simulink model "residual_FWD_INV_validation_v2"  (R2025a)
settings: Solver=VariableStepAuto  StartTime=0.0  StopTime=212  RelTol=1e-3
undefined symbols (not defined in the file or in its folder): National_Instruments, PCI, shadowInverseOptions, shadowOptions, shadowPressureOptions, singlePassOptions
libraries: sldrtlib x3
(part 1 of 2)
settings Model: Creator=dperera  LastModifiedBy=dperera

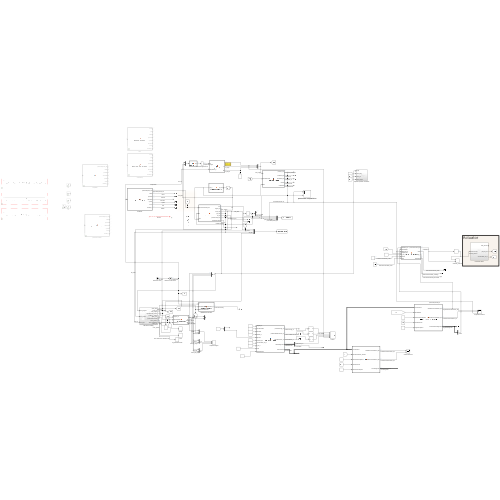
[thumbnail: Simulink's stored preview of the top-level diagram]
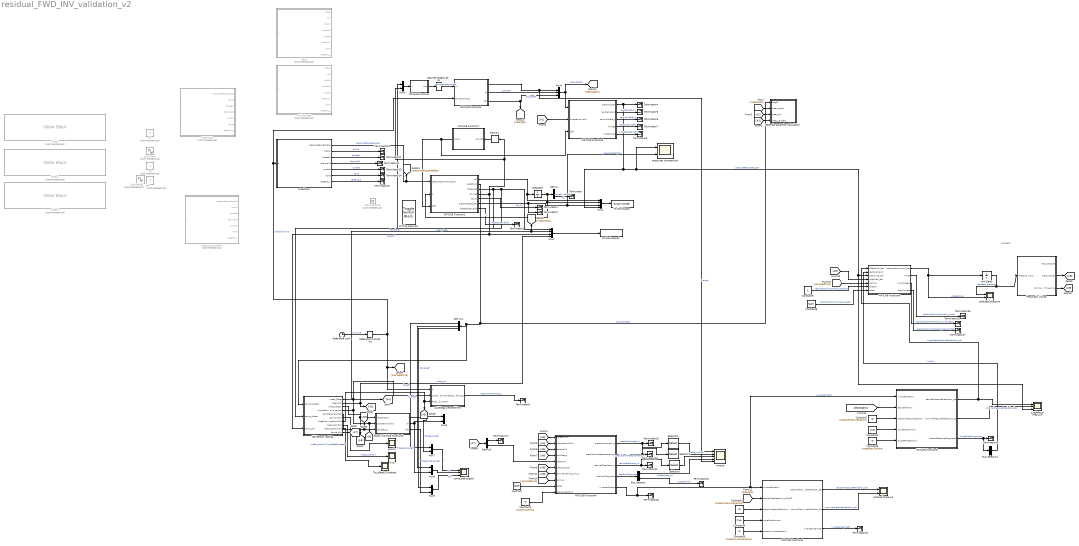
== system residual_FWD_INV_validation_v2 ==
  note: Actuator
  Bus Selector : BusSelector  OutputSignals=qMeasured_m,scoreValid
  Bus Selector1 : BusSelector  OutputSignals=valid
  Constant : Constant  Value=false  OutDataTypeStr=boolean
  Constant1 : Constant  Value=shadowOptions
  Constant2 : Constant  Value=shadowPressureOptions
  Constant3 : Constant  Value=shadowInverseOptions
  Constant4 : Constant  Value=true  OutDataTypeStr=boolean
  Constant5 : Constant  Value=true  OutDataTypeStr=boolean
  Constant6 : Constant  Value=singlePassOptions
  Constant7 : Constant  Value=shadowPressureOptions
  Constant8 : Constant  Value=false  OutDataTypeStr=boolean
  Constant9 : Constant
  Demux : Demux  Outputs=2
  Demux1 : Demux  Outputs=3
  Demux2 : Demux  Outputs=2
  Desired lengths 50 ms : ZeroOrderHold  SampleTime=0.05
  Integrator : Integrator  InitialCondition=[0;0;0;0]
  Inverse : Scope  NumInputPorts=5
      settings: ActiveDisplayYMinimum=-0.047306176084099816  ActiveDisplayYMaximum=0.024967148488830526  DataLoggingVariableName=ScopeData12
  MATLAB Function : MATLAB Function  TreatAsAtomicUnit=on
  MATLAB Function1 : MATLAB Function  TreatAsAtomicUnit=on
  MATLAB Function2 : MATLAB Function  TreatAsAtomicUnit=on
  MATLAB Function3 : MATLAB Function  TreatAsAtomicUnit=on
  MATLAB Function4 : MATLAB Function  TreatAsAtomicUnit=on
  MATLAB Function5 : MATLAB Function  TreatAsAtomicUnit=on
  MATLAB Function6 : MATLAB Function  TreatAsAtomicUnit=on
  MATLAB Function7 : MATLAB Function  TreatAsAtomicUnit=on
  MATLAB Function8 : MATLAB Function  TreatAsAtomicUnit=on
  MATLAB Function9 : MATLAB Function  TreatAsAtomicUnit=on
  Memory : Memory  InitialCondition=0.01
  Mux1 : Mux
  Mux2 : Mux
  Mux{3,5,7..9} (5 alike) : Mux  Inputs=2
  Mux6 : Mux  Inputs=3
  NDI Sensor reading : Subsystem
  P1 : Constant  Commented=on  Value=0
  P2 : Constant  Commented=on  Value=0
  P3 : Constant  Commented=on  Value=0
  Pneumatic Valves : Subsystem
  Reference clock : Clock
  Reference time 50 ms : ZeroOrderHold  SampleTime=0.05
  Selector1 : Selector  NumberOfDimensions=2  InputPortWidth=3  IndexOptions=Select all,Index vector (dialog)  Indices=[1 3],1  OutputSizes=1,1
  Selector2 : Selector  NumberOfDimensions=2  InputPortWidth=3  IndexOptions=Select all,Index vector (dialog)  Indices=[1 3],1  OutputSizes=1,1
  Selector3 : Selector  NumberOfDimensions=2  InputPortWidth=3  IndexOptions=Select all,Index vector (dialog)  Indices=[1 3],1  OutputSizes=1,1
  Seperate paramter calculation : Subsystem
  Sine Wave : Sin  Commented=on  Amplitude=1.5  Bias=1.5  Frequency=0.2  Phase=3*pi/2  SampleTime=0
  Sine Wave1 : Sin  Commented=on  Amplitude=1.5  Bias=1.5  Frequency=0.2  Phase=3*pi/2  SampleTime=0
  Slider : SliderBlock  Commented=on  ScaleMax=3
  Slider1 : SliderBlock  Commented=on  ScaleMax=3
  Slider2 : SliderBlock  Commented=on  ScaleMax=3
  Terminator{,1..15,17..27} (27 alike) : Terminator
  Terminator16 : Terminator  Commented=on
  Tip_offsetCOrrected : Scope
      settings: ActiveDisplayYMinimum=-0.22727653062343597  ActiveDisplayYMaximum=0.33693047368526458  DataLoggingVariableName=ScopeData9
  To Workspace : ToWorkspace  VariableName=dynamicModel  SaveFormat=Timeseries  SampleTime=-1
  To Workspace1 : ToWorkspace  VariableName=dynamic_NDI_meas_angle  SaveFormat=Timeseries  SampleTime=-1
  Unit Delay : UnitDelay  InitialCondition=[0;0;0]  SampleTime=0.05  HasFrameUpgradeWarning=on
  XYZ : Scope
      settings: ActiveDisplayYMinimum=-0.22727653062343597  ActiveDisplayYMaximum=0.33693047368526458  DataLoggingVariableName=ScopeData15
  circlesweep : MATLAB Function  Commented=on  TreatAsAtomicUnit=on
  computed lengths : Scope  NumInputPorts=3
      settings: ActiveDisplayYMinimum=-0.016802180124961048  ActiveDisplayYMaximum=0.019521084576218834  DataLoggingVariableName=ScopeData11
  gravity : Scope
      settings: ActiveDisplayYMinimum=-11.042014198482379  ActiveDisplayYMaximum=1.2784590278504426  DataLoggingVariableName=ScopeData10
  helix : MATLAB Function  Commented=on  TreatAsAtomicUnit=on
  kill the pressure : ToggleSwitchBlock
  pressure combine : MATLAB Function  Commented=on  TreatAsAtomicUnit=on
  pressures comparision : Scope  NumInputPorts=2
      settings: ActiveDisplayYMinimum=-0.37499999999999989  ActiveDisplayYMaximum=3.375  DataLoggingVariableName=ScopeData6
  residual Pressure : Scope  NumInputPorts=2
      settings: ActiveDisplayYMinimum=-0.44669940616060977  ActiveDisplayYMaximum=0.544979494551485  DataLoggingVariableName=ScopeData14
  selected_pressure : Scope  NumInputPorts=2
      settings: ActiveDisplayYMinimum=-0.37499999999999994  ActiveDisplayYMaximum=3.3750000000000004  DataLoggingVariableName=ScopeData17
  sineWave : MATLAB Function  TreatAsAtomicUnit=on
  singlePassl Pressure : Scope  NumInputPorts=3
      settings: ActiveDisplayYMinimum=-1.0880434782608694  ActiveDisplayYMaximum=2.9119565217391306  DataLoggingVariableName=ScopeData16
  stepWave : MATLAB Function  Commented=on  TreatAsAtomicUnit=on
  validMeasurementTime : MATLAB Function  TreatAsAtomicUnit=on
  wires:
  MATLAB Function1/1(dX) -> Mux1/1, Integrator/1  "dX"
  Integrator/1 -> MATLAB Function1/2(X), Mux1/2, Demux/1  "X"
  Demux/2 -> Terminator/1  "length velocity"
  MATLAB Function1/5(tau_N) -> Terminator1/1  "tau_N"
  MATLAB Function1/6(pressureUsed_bar) -> Terminator2/1, pressures comparision/2, Mux1/3  "pressureUsed_bar"
  MATLAB Function1/7(thetaObservable) -> Terminator3/1  "thetaObservable"
  Mux1/1 -> To Workspace/1
  Mux2/1 -> To Workspace1/1
  Mux6/1 -> MATLAB Function3/1(l), [deslengths]  "des_lengths"
  [A1] -> MATLAB Function3/2(orientationValid)
  MATLAB Function3/2(tauDesired_N) -> Terminator5/1  "tauDesired_N"
  MATLAB Function3/3(tauAvailable_N) -> Terminator6/1  "tauAvailable_N"
  MATLAB Function3/4(limited) -> Terminator7/1  "pressureLimited"
  MATLAB Function3/5(modelValid) -> Terminator8/1  "inverseModelValid"
  MATLAB Function7/1(k_N_m) -> MATLAB Function3/3(stiff), MATLAB Function1/3(stiff)
  Memory/1 -> MATLAB Function7/1(phi_rad)
  NDI Sensor reading/5(pollStart_s_control) -> MATLAB Function5/3(pollStart_s), [A6]
  NDI Sensor reading/8(meas_position) -> XYZ/1  "meas_position"
  NDI Sensor reading/1(meas_theta) -> [meastheta], Mux2/2  "meas_theta"
  NDI Sensor reading/3(meas_length) -> MATLAB Function5/1(lengths3_m), [A3]
  NDI Sensor reading/4(orientationValid_control) -> [A4], MATLAB Function5/2(orientationValid), validMeasurementTime/2(orientationValid), [A1]
  NDI Sensor reading/2(meas_phi) -> [A2], Mux2/4  "meas_phi"
  MATLAB Function5/1(l) -> Mux7/2, Mux5/1  "fitered_length"
  Demux1/3 -> Mux9/1  "dd_length"
  NDI Sensor reading/7(baseOreintationValid) -> [A5], validMeasurementTime/3(baseOrientationValid)
  Demux1/1 -> Mux7/1  "length"
  Demux1/2 -> Mux8/1  "d_length"
  Mux8/1 -> computed lengths/2  "dl"
  MATLAB Function5/3(ddl) -> Mux9/2  "filtered_dd_length"
  Mux7/1 -> computed lengths/1  "l"
  MATLAB Function5/2(dl) -> Mux8/2, Mux5/2  "filtered_d_length"
  Mux9/1 -> computed lengths/3  "ddl"
  [A3] -> Seperate paramter calculation/4(meas_lengths)
  [A2] -> Seperate paramter calculation/3(meas_phi)
  Reference clock/1 -> Reference time 50 ms/1  "sim time"
  Reference time 50 ms/1 -> MATLAB Function2/2(sampleTime_s), sineWave/1(t), [sampledtime], validMeasurementTime/1(t)  "sampled time"
  MATLAB Function1/2(lengths_m) -> Seperate paramter calculation/1(length), NDI Sensor reading/1(comp_lengths), Demux1/1  "comp_lengths"
  validMeasurementTime/1(measurementTime_s) -> Terminator9/1  "measurementTime_s"
  sineWave/2(trialId) -> Terminator10/1  "trialId"
  sineWave/3(phaseId) -> Terminator11/1  "phaseId"
  sineWave/4(channelId) -> Terminator12/1  "channelId"
  sineWave/5(cycleId) -> Terminator13/1  "cycleId"
  sineWave/6(done) -> Terminator14/1  "done"
  sineWave/7(testEnd_s) -> Terminator15/1  "testEnd_s"
  ? -> Terminator16/1  "direction"
  MATLAB Function/1(lout) -> Desired lengths 50 ms/1
  Desired lengths 50 ms/1 -> MATLAB Function2/1(lIn)  "sampled des_length"
  Mux3/1 -> MATLAB Function/1(u)
  MATLAB Function2/1(l) -> Inverse/5, Mux6/1  "length"
  MATLAB Function2/2(dl) -> Mux6/2  "d_length"
  MATLAB Function2/3(ddl) -> Mux6/3, [ddlength]  "dd_length"
  [meastheta] -> Seperate paramter calculation/2(meas_theta)
  NDI Sensor reading/9(meas_positionTip) -> Tip_offsetCOrrected/1  "meas_positionTip_offsetCorrected"
  NDI Sensor reading/6(gravity_arm) -> gravity/1
  MATLAB Function3/1(pressure_bar) -> Mux1/4, pressures comparision/1, MATLAB Function9/3(pNominal_bar), singlePassl Pressure/3, Terminator4/1  "pressureRequested_bar"
  [A3] -> MATLAB Function4/1(lengths3_m)
  [A4] -> MATLAB Function4/2(orientationValid)
  [A5] -> MATLAB Function4/3(baseValid)
  [A6] -> MATLAB Function4/4(pollStart_s)
  Demux2/2 -> MATLAB Function4/5(tipFrame)
  NDI Sensor reading/10(frame_out) -> [A7]
  [A7] -> Demux2/1
  Demux2/1 -> Terminator17/1
  [A8] -> MATLAB Function4/6(pressure_bar)
  [sampledtime] -> MATLAB Function4/8(t_sim_s)
  Constant/1 -> MATLAB Function4/9(reset)
  Constant1/1 -> MATLAB Function4/10(shadowOptions)
  Pneumatic Valves/2(pressure_bar) -> [A8]
  Pneumatic Valves/3(commandTime_sim_s) -> [A9]
  [A9] -> MATLAB Function4/7(commandTime_sim_s)
  MATLAB Function4/4(shadowDiagnostic) -> Bus Selector/1  "shadowDiagnotic"
  MATLAB Function4/5(inverseContext) -> MATLAB Function8/1(inverseContext), MATLAB Function6/1(inverseContext), Terminator18/1  "inverseContext"
  MATLAB Function4/1(predictionLength_m) -> Selector2/1, Terminator19/1  "predictionLength_m"
  MATLAB Function4/2(predictionAtMeasurement_m) -> Selector1/1, Terminator20/1  "predictionAtMeasurement_m"
  MATLAB Function4/3(retimedPrediction_m) -> Selector3/1, Terminator21/1  "retimePrediction_m"
  Bus Selector/1 -> Inverse/4  "<qMeasured_m>"
  Selector1/1 -> Inverse/2  "pred_withNDI"
  Bus Selector/2 -> Terminator22/1  "<scoreValid>"
  MATLAB Function1/3(theta_rad) -> NDI Sensor reading/2(comp_ltheta), Mux3/1, Mux2/1  "des_theta"
  MATLAB Function1/4(phi_rad) -> NDI Sensor reading/3(comp_phi), Mux2/3, Mux3/2, Memory/1  "des_phi"
  Selector2/1 -> Inverse/1
  Selector3/1 -> Inverse/3
  [ddlength] -> MATLAB Function6/2(desiredAcceleration_mPerS2)
  Constant2/1 -> MATLAB Function6/3(shadowPressureOptions)
  Constant3/1 -> MATLAB Function6/5(shadowInverseOptions)
  Constant4/1 -> MATLAB Function6/4(variableCommon)
  MATLAB Function6/3(inverseDiagnostic) -> Terminator23/1  "inverseDiagnostic"
  MATLAB Function6/1(residualPressurePrediction_bar) -> residual Pressure/1  "residualPressurePrediction_bar"
  MATLAB Function6/2(nominalPressurePrediction_bar) -> residual Pressure/2  "nominalPressurePrediction_bar"
  Constant5/1 -> MATLAB Function8/4(variableCommon)
  Constant6/1 -> MATLAB Function8/5(singlePassOptions)
  Constant7/1 -> MATLAB Function8/3(shadowPressureOptions)
  MATLAB Function8/3(desiredPressureDiagnostic) -> Bus Selector1/1, Terminator24/1  "singlePassDiagnostic"
  MATLAB Function8/1(desiredPressurePrediction_bar) -> MATLAB Function9/1(pResidual_bar), singlePassl Pressure/1  "singlePassPressurePrediction_bar"
  MATLAB Function8/2(nominalPressurePrediction_bar) -> singlePassl Pressure/2  "nominalPressurePrediction_bar"
  [deslengths] -> MATLAB Function8/2(desiredMotion)
  MATLAB Function9/1(pressureCommand_bar) -> Unit Delay/1, selected_pressure/2  "useResidual"
  Unit Delay/1 -> selected_pressure/1, Pneumatic Valves/1(Pressure input)  "selected_pressure"
  Bus Selector1/1 -> MATLAB Function9/2(residualValid)  "<valid>"
  sineWave/1(pressureRequest_bar) -> MATLAB Function1/1(pressureCommand_bar), [pressureRequestedbar]  "pressureRequested_bar"
  [A8] -> MATLAB Function9/4(pApplied_bar)
  [sampledtime] -> MATLAB Function9/5(t_sim_s)
  Constant8/1 -> MATLAB Function9/7(reset)  "residualCommandValid_reset"
  Constant9/1 -> MATLAB Function9/6(enable)  "residualCommandValid_enable"
  MATLAB Function9/2(mode) -> Terminator25/1  "residualCommandValid_mode"
  MATLAB Function9/3(invalidAge_s) -> Terminator26/1  "residualCommandValid_invalidAge"
  MATLAB Function9/4(slewLimited) -> Terminator27/1  "residualCommandValid_slewLimited"

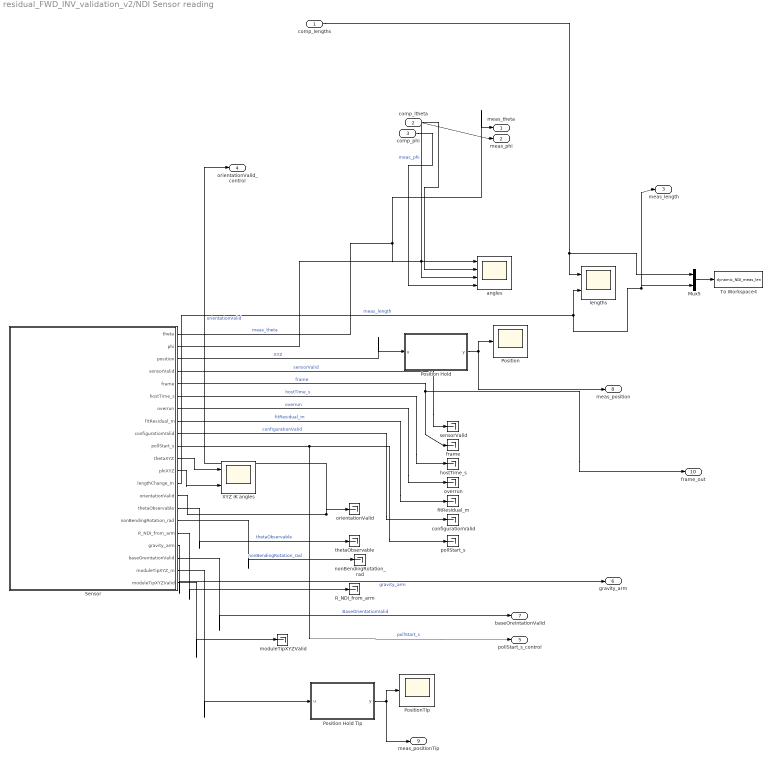
== system residual_FWD_INV_validation_v2/NDI Sensor reading ==
  comp_lengths : Inport
  comp_ltheta : Inport  Port=2
  comp_phi : Inport  Port=3
  Mux5 : Mux  Inputs=2
  Position : Scope
      settings: ActiveDisplayYMinimum=-0.21656345474719998  ActiveDisplayYMaximum=0.33777835857868188
  Position Hold : MATLAB Function  TreatAsAtomicUnit=on
  Position Hold Tip : MATLAB Function  TreatAsAtomicUnit=on
  PositionTip : Scope
      settings: ActiveDisplayYMinimum=-0.21656345474719998  ActiveDisplayYMaximum=0.33777835857868188  DataLoggingVariableName=ScopeData8
  R_NDI_from_arm : Terminator
  Sensor : Subsystem
  To Workspace4 : ToWorkspace  VariableName=dynamic_NDI_meas_len  SaveFormat=Timeseries  SampleTime=-1
  XYZ IK angles : Scope  NumInputPorts=2
      settings: DataLoggingVariableName=ScopeData2
  angles : Scope  NumInputPorts=4
      settings: ActiveDisplayYMinimum=-3.9269908169872414  ActiveDisplayYMaximum=3.9269908169872414
  configurationValid : Terminator
  fitResidual_m : Terminator
  frame : Terminator
  hostTime_s : Terminator
  lengths : Scope  NumInputPorts=2
      settings: ActiveDisplayYMinimum=-0.0017146774565175815  ActiveDisplayYMaximum=0.0020057370608089205  DataLoggingVariableName=ScopeData3
  moduleTipXYZValid : Terminator
  nonBendingRotation_rad : Terminator
  orientationValid : Terminator
  overrun : Terminator
  pollStart_s : Terminator
  sensorValid : Terminator
  thetaObservable : Terminator
  meas_theta : Outport
  meas_phi : Outport  Port=2
  meas_length : Outport  Port=3
  orientationValid_control : Outport  Port=4
  pollStart_s_control : Outport  Port=5
  gravity_arm : Outport  Port=6
  baseOreintationValid : Outport  Port=7
  meas_position : Outport  Port=8
  meas_positionTip : Outport  Port=9
  frame_out : Outport  Port=10
  wires:
  Sensor/13(lengthChange_m) -> lengths/2, meas_length/1, Mux5/2  "meas_length"
  comp_lengths/1 -> lengths/1, Mux5/1
  Sensor/10(pollStart_s) -> pollStart_s_control/1, pollStart_s/1  "pollStart_s"
  Sensor/2(phi) -> angles/3, meas_phi/1  "meas_phi"
  Sensor/3(position) -> Position Hold/1(u)  "XYZ"
  Sensor/1(theta) -> meas_theta/1, angles/1  "meas_theta"
  Sensor/6(hostTime_s) -> hostTime_s/1  "hostTIme_s"
  Sensor/9(configurationValid) -> configurationValid/1  "configurationValid"
  Sensor/4(sensorValid) -> sensorValid/1  "sensorValid"
  Sensor/7(overrun) -> overrun/1  "overrun"
  Sensor/5(frame) -> frame_out/1, frame/1  "frame"
  comp_ltheta/1 -> angles/2
  Sensor/8(fitResidual_m) -> fitResidual_m/1  "fitResidual_m"
  Sensor/12(phiXYZ) -> XYZ IK angles/2
  Sensor/11(thetaXYZ) -> XYZ IK angles/1
  Position Hold/1(y) -> Position/1, meas_position/1
  Mux5/1 -> To Workspace4/1
  Sensor/14(orientationValid) -> orientationValid_control/1, orientationValid/1  "orientationValid"
  Sensor/16(nonBendingRotation_rad) -> nonBendingRotation_rad/1  "nonBendingRotation_rad"
  Sensor/15(thetaObservable) -> thetaObservable/1  "thetaObservable"
  comp_phi/1 -> angles/4
  Sensor/19(baseOreintationValid) -> baseOreintationValid/1  "BaseOrientationValid"
  Sensor/17(R_NDI_from_arm) -> R_NDI_from_arm/1
  Sensor/18(gravity_arm) -> gravity_arm/1  "gravity_arm"
  Sensor/20(moduleTipXYZ_m) -> Position Hold Tip/1(u)
  Position Hold Tip/1(y) -> meas_positionTip/1, PositionTip/1
  Sensor/21(moduleTipXYZValid) -> moduleTipXYZValid/1

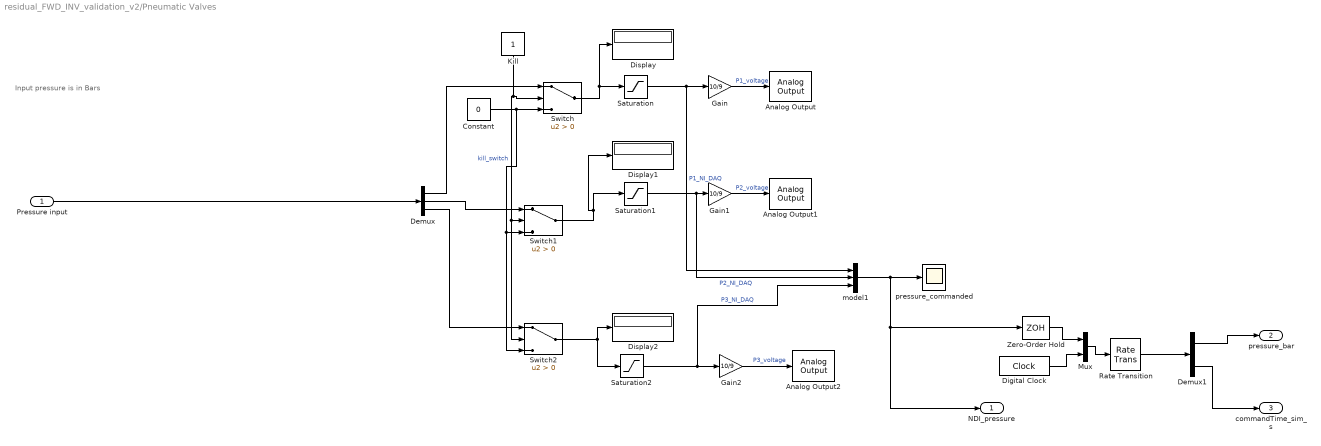
== system residual_FWD_INV_validation_v2/Pneumatic Valves ==
  note: Input pressure is in Bars
  Pressure input : Inport
  Analog Output : sldrtlib/Analog Output  SampleTime=1/100  MaxMissedTicks=inf  ShowMissedTicks=off  YieldWhenWaiting=off  DrvName=National_Instruments/PCI-6703  DrvAddress=4294967295  DrvOptions=0  Channels=1  RangeMode=1  VoltRange=1  InitialValue=0  FinalValue=0
      settings: AttributesFormatString=National Instruments\nPCI-6703 [auto]
  Analog Output1 : sldrtlib/Analog Output  SampleTime=1/100  MaxMissedTicks=inf  ShowMissedTicks=off  YieldWhenWaiting=off  DrvName=National_Instruments/PCI-6703  DrvAddress=4294967295  DrvOptions=0  Channels=2  RangeMode=1  VoltRange=1  InitialValue=0  FinalValue=0
      settings: AttributesFormatString=National Instruments\nPCI-6703 [auto]
  Analog Output2 : sldrtlib/Analog Output  SampleTime=1/100  MaxMissedTicks=inf  ShowMissedTicks=off  YieldWhenWaiting=off  DrvName=National_Instruments/PCI-6703  DrvAddress=4294967295  DrvOptions=0  Channels=3  RangeMode=1  VoltRange=1  InitialValue=0  FinalValue=0
      settings: AttributesFormatString=National Instruments\nPCI-6703 [auto]
  Constant : Constant  Value=0
  Demux : Demux  Outputs=3
  Demux1 : Demux  Outputs=[3 1]
  Digital Clock : DigitalClock  SampleTime=0.01
  Display : Display
  Display1 : Display
  Display2 : Display
  Gain : Gain  Gain=10/9
  Gain1 : Gain  Gain=10/9
  Gain2 : Gain  Gain=10/9
  Kill : Constant
  Mux : Mux  Inputs=2
  Rate Transition : RateTransition  InitialCondition=[0]  OutPortSampleTime=0.05
  Saturation : Saturate  UpperLimit=3  LowerLimit=0
  Saturation1 : Saturate  UpperLimit=3  LowerLimit=0
  Saturation2 : Saturate  UpperLimit=3  LowerLimit=0
  Switch : Switch  Criteria=u2 > Threshold  SaturateOnIntegerOverflow=off  InputSameDT=off
  Switch1 : Switch  Criteria=u2 > Threshold  SaturateOnIntegerOverflow=off  InputSameDT=off
  Switch2 : Switch  Criteria=u2 > Threshold  SaturateOnIntegerOverflow=off  InputSameDT=off
  Zero-Order Hold : ZeroOrderHold  SampleTime=0.01
  model1 : Mux  Inputs=3
  pressure_commanded : Scope
      settings: ActiveDisplayYMinimum=-0.37499999999999989  ActiveDisplayYMaximum=3.375  DataLoggingVariableName=ScopeData7
  NDI_pressure : Outport
  pressure_bar : Outport  Port=2
  commandTime_sim_s : Outport  Port=3
  wires:
  Constant/1 -> Switch2/3, Switch1/3, Switch/3
  Kill/1 -> Switch2/2, Switch1/2, Switch/2  "kill_switch"
  Switch/1 -> Display/1, Saturation/1
  Gain/1 -> Analog Output/1  "P1_voltage"
  Saturation/1 -> model1/1, Gain/1  "P1_NI_DAQ"
  Demux/3 -> Switch2/1
  Gain1/1 -> Analog Output1/1  "P2_voltage"
  Gain2/1 -> Analog Output2/1  "P3_voltage"
  Saturation2/1 -> model1/3, Gain2/1  "P3_NI_DAQ"
  Switch2/1 -> Saturation2/1, Display2/1
  Demux/2 -> Switch1/1
  Switch1/1 -> Saturation1/1, Display1/1
  model1/1 -> NDI_pressure/1, Zero-Order Hold/1, pressure_commanded/1
  Saturation1/1 -> model1/2, Gain1/1  "P2_NI_DAQ"
  Demux/1 -> Switch/1
  Pressure input/1 -> Demux/1
  Zero-Order Hold/1 -> Mux/1
  Digital Clock/1 -> Mux/2
  Mux/1 -> Rate Transition/1
  Rate Transition/1 -> Demux1/1
  Demux1/1 -> pressure_bar/1
  Demux1/2 -> commandTime_sim_s/1

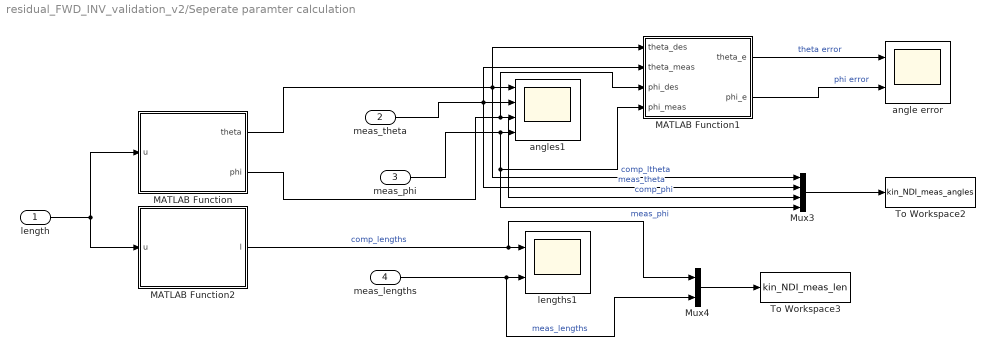
== system residual_FWD_INV_validation_v2/Seperate paramter calculation ==
  length : Inport
  meas_theta : Inport  Port=2
  meas_phi : Inport  Port=3
  meas_lengths : Inport  Port=4
  MATLAB Function : MATLAB Function  TreatAsAtomicUnit=on
  MATLAB Function1 : MATLAB Function  TreatAsAtomicUnit=on
  MATLAB Function2 : MATLAB Function  TreatAsAtomicUnit=on
  Mux3 : Mux
  Mux4 : Mux  Inputs=2
  To Workspace2 : ToWorkspace  VariableName=kin_NDI_meas_angles  SaveFormat=Timeseries  SampleTime=-1
  To Workspace3 : ToWorkspace  VariableName=kin_NDI_meas_len  SaveFormat=Timeseries  SampleTime=-1
  angle error : Scope  NumInputPorts=2
      settings: ActiveDisplayYMinimum=-3.908241267522468  ActiveDisplayYMaximum=3.9243412430226807  DataLoggingVariableName=ScopeData13
  angles1 : Scope  NumInputPorts=4
      settings: ActiveDisplayYMinimum=-3.9269137322662839  ActiveDisplayYMaximum=3.9265599408279468  DataLoggingVariableName=ScopeData4
  lengths1 : Scope  NumInputPorts=2
      settings: ActiveDisplayYMinimum=-0.02243223759551808  ActiveDisplayYMaximum=0.037530111947788623  DataLoggingVariableName=ScopeData5
  wires:
  meas_lengths/1 -> Mux4/2, lengths1/2  "meas_lengths"
  meas_theta/1 -> MATLAB Function1/2(theta_meas), Mux3/2, angles1/2  "meas_theta"
  MATLAB Function/2(phi) -> MATLAB Function1/3(phi_des), Mux3/3, angles1/3  "comp_phi"
  Mux3/1 -> To Workspace2/1
  meas_phi/1 -> MATLAB Function1/4(phi_meas), Mux3/4, angles1/4  "meas_phi"
  MATLAB Function/1(theta) -> MATLAB Function1/1(theta_des), Mux3/1, angles1/1  "comp_ltheta"
  Mux4/1 -> To Workspace3/1
  MATLAB Function2/1(l) -> Mux4/1, lengths1/1  "comp_lengths"
  length/1 -> MATLAB Function2/1(u), MATLAB Function/1(u)
  MATLAB Function1/1(theta_e) -> angle error/1  "theta error"
  MATLAB Function1/2(phi_e) -> angle error/2  "phi error"

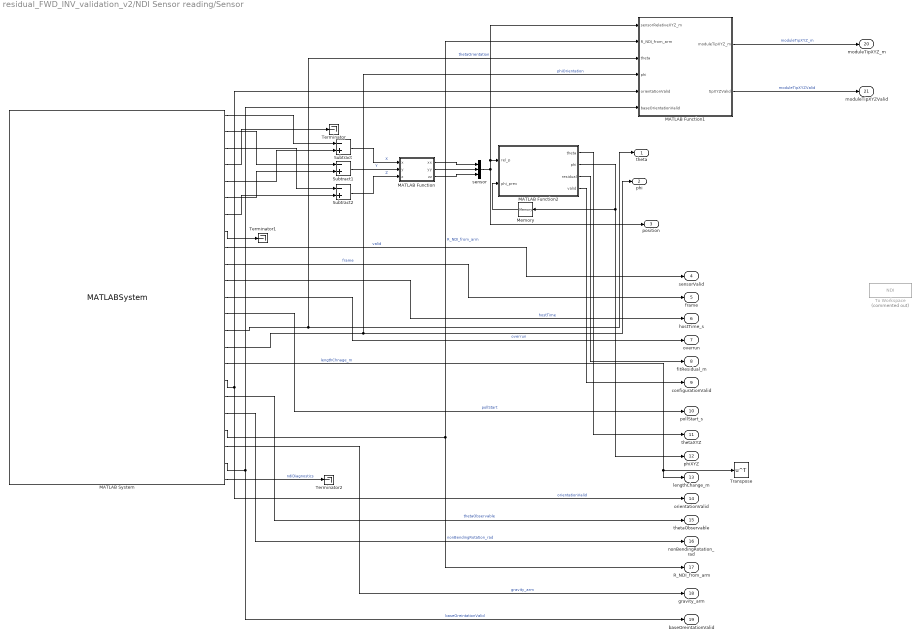
== system residual_FWD_INV_validation_v2/NDI Sensor reading/Sensor ==
  MATLAB Function : MATLAB Function  TreatAsAtomicUnit=on
  MATLAB Function1 : MATLAB Function  TreatAsAtomicUnit=on
  MATLAB Function2 : MATLAB Function  TreatAsAtomicUnit=on
  MATLAB System : MATLABSystem  System=AuroraReader_s2_BaseRotation  Port=COM12  BaudRate=921600  SamplePeriod=0.05  BaseSensorId=0A  TipSensorId=0B  CalibrationFile=C:\Users\dperera\OneDrive - Texas A&M University\Lab\Research\fDyn_ExpCom\hyDyn_Ctrl\ndi_orientation_recordings\calibration_20260930_190505_898.mat  PreflightSeconds=5  ActuatorRadius=0.013  ReferenceGravity_arm=[ 0; 0; -9.81 ]  SimulateUsing=Interpreted execution
      mask Type: AuroraReader_s2_BaseRotation
  Memory : Memory  InitialCondition=0.0001
  Subtract : Sum  Inputs=-+
  Subtract1 : Sum  Inputs=-+
  Subtract2 : Sum  Inputs=-+
  Terminator : Terminator
  Terminator1 : Terminator
  Terminator2 : Terminator
  To Workspace : ToWorkspace  Commented=on  VariableName=NDI  SaveFormat=Timeseries  SampleTime=-1
  Transpose : Math  Operator=transpose
  sensor : Mux  Inputs=3
  theta : Outport
  phi : Outport  Port=2
  position : Outport  Port=3
  sensorValid : Outport  Port=4
  frame : Outport  Port=5
  hostTime_s : Outport  Port=6
  overrun : Outport  Port=7
  fitResidual_m : Outport  Port=8
  configurationValid : Outport  Port=9
  pollStart_s : Outport  Port=10
  thetaXYZ : Outport  Port=11
  phiXYZ : Outport  Port=12
  lengthChange_m : Outport  Port=13
  orientationValid : Outport  Port=14
  thetaObservable : Outport  Port=15
  nonBendingRotation_rad : Outport  Port=16
  R_NDI_from_arm : Outport  Port=17
  gravity_arm : Outport  Port=18
  baseOreintationValid : Outport  Port=19
  moduleTipXYZ_m : Outport  Port=20
  moduleTipXYZValid : Outport  Port=21
  wires:
  MATLAB System/2 -> Subtract1/1
  MATLAB Function/3(zz) -> sensor/3
  Subtract1/1 -> MATLAB Function/2(y)  "Y"
  Subtract2/1 -> MATLAB Function/3(z)  "Z"
  MATLAB System/5 -> Subtract/2
  sensor/1 -> MATLAB Function1/1(sensorRelativeXYZ_m), MATLAB Function2/1(rel_p), position/1
  MATLAB System/8 -> Terminator1/1
  MATLAB Function/1(xx) -> sensor/1
  Subtract/1 -> MATLAB Function/1(x)  "X"
  MATLAB Function/2(yy) -> sensor/2
  MATLAB System/1 -> Subtract/1
  MATLAB Function2/2(phi) -> Memory/1, phiXYZ/1
  MATLAB System/7 -> Subtract2/2
  MATLAB System/4 -> Terminator/1
  MATLAB System/3 -> Subtract2/1
  MATLAB System/6 -> Subtract1/2
  Memory/1 -> MATLAB Function2/2(phi_prev)
  MATLAB System/9 -> sensorValid/1  "valid"
  MATLAB System/11 -> hostTime_s/1  "hostTime"
  MATLAB System/12 -> overrun/1  "overrun"
  MATLAB Function2/3(residual) -> fitResidual_m/1
  MATLAB Function2/4(valid) -> configurationValid/1
  MATLAB System/13 -> pollStart_s/1  "pollStart"
  MATLAB System/14 -> MATLAB Function1/3(theta), theta/1  "thetaOrientation"
  MATLAB System/15 -> MATLAB Function1/4(phi), phi/1  "phiOrientation"
  MATLAB Function2/1(theta) -> thetaXYZ/1
  MATLAB System/16 -> lengthChange_m/1, Transpose/1  "lengthChnage_m"
  MATLAB System/17 -> orientationValid/1, MATLAB Function1/5(orientationValid)  "orientationValid"
  MATLAB System/18 -> thetaObservable/1  "thetaObservable"
  MATLAB System/19 -> nonBendingRotation_rad/1  "nonBendingRotation_rad"
  MATLAB System/10 -> frame/1  "frame"
  MATLAB System/20 -> R_NDI_from_arm/1, MATLAB Function1/2(R_NDI_from_arm)  "R_NDI_from_arm"
  MATLAB System/21 -> gravity_arm/1  "gravity_arm"
  MATLAB System/22 -> baseOreintationValid/1, MATLAB Function1/6(baseOrientationValid)  "baseOreintationValid"
  MATLAB Function1/1(moduleTipXYZ_m) -> moduleTipXYZ_m/1  "moduleTipXYZ_m"
  MATLAB Function1/2(tipXYZValid) -> moduleTipXYZValid/1  "moduleTipXYZValid"
  MATLAB System/23 -> Terminator2/1  "ndiDiagnostics"

== matlab function residual_FWD_INV_validation_v2/validMeasurementTime ==
  data: t input; measurementTime_s output; orientationValid input; baseOrientationValid input
function measurementTime_s = validMeasurementTime( ...
    t, orientationValid, baseOrientationValid)
%#codegen

persistent lastValidTime
if isempty(lastValidTime)
    lastValidTime = -1.0;
end

if orientationValid && baseOrientationValid && isfinite(t)
    lastValidTime = t;
end

measurementTime_s = lastValidTime;
end

== matlab function residual_FWD_INV_validation_v2/NDI Sensor reading/Position Hold Tip ==
  data: u input; y output
function y = fcn(u)
persistent lastPosition
if isempty(lastPosition), lastPosition=nan(3,1); end
if all(isfinite(u)), lastPosition=u; end
y=lastPosition;
end

== matlab function residual_FWD_INV_validation_v2/MATLAB Function5 ==
  data: lengths3_m input; l output; dl output; ddl output; orientationValid input; pollStart_s input
function [l, dl, ddl] = filteredDerivatives(lengths3_m, orientationValid, pollStart_s)
%#codegen
% NDI lengths are [l1;l2;l3]; model coordinates are [l2;l3].
% Invalid or repeated BX frames do not update the derivative states.
persistent lastL lastT velocity acceleration
if isempty(lastT)
    lastL = nan(2,1);
    lastT = -1;
    velocity = zeros(2,1);
    acceleration = zeros(2,1);
end
l = lastL;
dl = velocity;
ddl = acceleration;
if ~orientationValid || ~all(isfinite(lengths3_m)) || ~isfinite(pollStart_s)
    return;
end
q = [lengths3_m(2); lengths3_m(3)];
if lastT < 0
    lastL = q;
    lastT = pollStart_s;
    l = q;
    return;
end
dt = pollStart_s-lastT;
if dt > 1e-6
    rawVelocity = (q-lastL)/dt;
    oldVelocity = velocity;
    alphaV = dt/(0.20+dt);
    velocity = velocity + alphaV*(rawVelocity-velocity);
    rawAcceleration = (velocity-oldVelocity)/dt;
    alphaA = dt/(0.30+dt);
    acceleration = acceleration + alphaA*(rawAcceleration-acceleration);
    lastL = q;
    lastT = pollStart_s;
end
l = lastL;
dl = velocity;
ddl = acceleration;
end

== matlab function residual_FWD_INV_validation_v2/sineWave ==
  data: t input; pressureRequest_bar output; trialId output; phaseId output; channelId output; cycleId output; done output; testEnd_s output
function [pressureRequest_bar,trialId,phaseId,channelId,cycleId,done,testEnd_s] = rlPressureSineBlock(t)
%#codegen
% OPEN-LOOP raw pressure request: peak/2*(1-cos(omega*time)).
% channelSelection: 1=P1, 2=P2, 3=P3, 0=all three separately.
channelSelection=0;
peak_bar=3.0;
omega_radPerS=0.8;
cyclesPerTrial=3;
repeats=2;
initialZero_s=5.0;
relax_s=10.0;
% phase: -1 invalid time, 0 initial zero, 4 zero relaxation,
% 5 periodic excitation, 9 complete. Cycles join at zero with zero slope.
assert(channelSelection>=0 && channelSelection<=3 && channelSelection==floor(channelSelection));
assert(peak_bar>=0 && peak_bar<=3 && omega_radPerS>0);
assert(cyclesPerTrial>=1 && cyclesPerTrial==floor(cyclesPerTrial));
assert(repeats>=1 && repeats==floor(repeats) && initialZero_s>=0 && relax_s>0);
nChannels=1;if channelSelection==0,nChannels=3;end
period_s=2*pi/omega_radPerS;
excitation_s=cyclesPerTrial*period_s;
trialDuration_s=excitation_s+relax_s;
nTrials=nChannels*repeats;
testEnd_s=initialZero_s+nTrials*trialDuration_s;
pressureRequest_bar=zeros(3,1);trialId=0;phaseId=0;channelId=0;cycleId=0;done=false;
if ~isfinite(t) || t<0,phaseId=-1;return;end
if t<initialZero_s,return;end
if t>=testEnd_s,phaseId=9;done=true;return;end
index=floor((t-initialZero_s)/trialDuration_s);
trialId=index+1;channelId=channelSelection;
if channelSelection==0,channelId=floor(index/repeats)+1;end
local=t-initialZero_s-index*trialDuration_s;
if local<excitation_s
    phaseId=5;cycleId=floor(local/period_s)+1;
    pressureRequest_bar(channelId)=peak_bar*.5*(1-cos(omega_radPerS*local));
else
    phaseId=4;
end
end

== matlab function residual_FWD_INV_validation_v2/MATLAB Function7 ==
  data: phi_rad input; k_N_m output
function k_N_m = stiffnessFromPhiBlock(phi_rad)
%#codegen
% Scalar P1 effective stiffness from the 2026-10-02 fitted data (N/m).
% Input may be current phi or externally delayed phi, in radians.
% Endpoint extension: <=0.09425 rad -> 4132; >=2.05594 rad -> 953.333.
% Invalid input uses the near-straight endpoint (not a sensor-validity gate).
breaks = [0.094252336020426999 0.31719551885716302 ...
          0.84254655402063705 1.3628983100343199 ...
          1.7568402609821301 2.0559364288348001];
coefs = [-301.18295127845971 -90.779050026315701 -3508.295263988015 4132; ...
          8648.306884889811 -4672.8276757423591 -3593.6820922138418 3342; ...
          222.76060985869111 882.71017208803505 -1342.7968944369923 1418.3333333333301; ...
          341.14621515352195 107.09908322703643 -243.20935379879649 990; ...
          254.06580436465293 166.20780898136815 0 931.66666666666697];
if ~isfinite(phi_rad) || phi_rad <= breaks(1)
    k_N_m = 4132;
    return;
end
if phi_rad >= breaks(6)
    k_N_m = 953.333333333333;
    return;
end
segment = 1;
for j = 2:5
    if phi_rad >= breaks(j), segment = j; end
end
x = phi_rad-breaks(segment);
k_N_m = ((coefs(segment,1)*x+coefs(segment,2))*x ...
           +coefs(segment,3))*x+coefs(segment,4);
end

== matlab function residual_FWD_INV_validation_v2/stepWave ==
  data: t input; pressureRequest_bar output; trialId output; phaseId output; channelId output; cycleId output; done output; testEnd_s output
function [pressureRequest_bar,trialId,phaseId,channelId,cycleId,done,testEnd_s] = rlPressureStepsBlock(t)
%#codegen
% OPEN-LOOP REQUEST ONLY. Connect through the existing Kill/pressure limits.
% channelSelection: 1=P1, 2=P2, 3=P3, 0=all three tested separately.
channelSelection=0;
peakLevels_bar=[1.0 2.0 3.0];
repeats=2;
initialZero_s=5.0;
rise_s=3.0;
hold_s=10.0;
fall_s=3.0;
relax_s=10.0;
% phase: -1 invalid time, 0 initial zero, 1 rise, 2 hold, 3 fall,
% 4 zero relaxation, 9 complete. No deadzone subtraction.
assert(channelSelection>=0 && channelSelection<=3 && channelSelection==floor(channelSelection));
assert(repeats>=1 && repeats==floor(repeats));
assert(all(peakLevels_bar>=0 & peakLevels_bar<=3));
assert(initialZero_s>=0 && rise_s>0 && hold_s>0 && fall_s>0 && relax_s>0);
nChannels=1;if channelSelection==0,nChannels=3;end
nLevels=numel(peakLevels_bar);
trialDuration_s=rise_s+hold_s+fall_s+relax_s;
nTrials=nChannels*repeats*nLevels;
testEnd_s=initialZero_s+nTrials*trialDuration_s;
pressureRequest_bar=zeros(3,1);trialId=0;phaseId=0;channelId=0;cycleId=0;done=false;
if ~isfinite(t) || t<0,phaseId=-1;return;end
if t<initialZero_s,return;end
if t>=testEnd_s,phaseId=9;done=true;return;end
index=floor((t-initialZero_s)/trialDuration_s);
trialId=index+1;
channelId=channelSelection;
if channelSelection==0,channelId=floor(index/(repeats*nLevels))+1;end
cycleId=mod(floor(index/nLevels),repeats)+1;
level=mod(index,nLevels)+1;
local=t-initialZero_s-index*trialDuration_s;
peak=peakLevels_bar(level);
if local<rise_s
    phaseId=1;u=local/rise_s;p=peak*u*u*(3-2*u);
elseif local<rise_s+hold_s
    phaseId=2;p=peak;
elseif local<rise_s+hold_s+fall_s
    phaseId=3;u=(local-rise_s-hold_s)/fall_s;p=peak*(1-u*u*(3-2*u));
else
    phaseId=4;p=0;
end
pressureRequest_bar(channelId)=p;
end

== matlab function residual_FWD_INV_validation_v2/circlesweep ==
  data: t input; theta output; phi output; trialId output; phaseId output; cycleId output; direction output; done output; testEnd_s output
function [theta,phi,trialId,phaseId,cycleId,direction,done,testEnd_s] = rlCircleSweepReferenceBlock(t)
%#codegen
% Requested ANGLES, not pressures or measured arm motion.
% Five phi levels, five circles each, no pauses between revolutions.
phiLevels_rad=[0.2 0.8 1.0 1.5 2.5];
circleTime_s=10.0;
circlesPerTrial=5;
initialZero_s=5.0;
phiRise_s=5.0;
targetWait_s=3.0;
phiFall_s=5.0;
zeroHold_s=10.0;
rotationDirection=1; % +1 or -1; keep unwrapped theta for downstream rates.
% phase: -1 invalid,0 baseline,1 phi rise,2 target wait,3 phi fall,
% 4 zero hold,5 circles,9 complete.
assert(all(phiLevels_rad>=0 & phiLevels_rad<=pi));
assert(circleTime_s>0 && circlesPerTrial>=1 && circlesPerTrial==floor(circlesPerTrial));
assert(phiRise_s>0 && phiFall_s>0 && targetWait_s>=0 && zeroHold_s>=0 && initialZero_s>=0);
assert(abs(rotationDirection)==1);
circleDuration_s=circlesPerTrial*circleTime_s;
trialDuration_s=phiRise_s+targetWait_s+circleDuration_s+phiFall_s+zeroHold_s;
nTrials=numel(phiLevels_rad);
testEnd_s=initialZero_s+nTrials*trialDuration_s;
theta=0;phi=0;trialId=0;phaseId=0;cycleId=0;direction=0;done=false;
if ~isfinite(t) || t<0,phaseId=-1;return;end
if t<initialZero_s,return;end
if t>=testEnd_s
    theta=rotationDirection*2*pi*circlesPerTrial*nTrials;
    phaseId=9;done=true;return;
end
index=floor((t-initialZero_s)/trialDuration_s);
trialId=index+1;
local=t-initialZero_s-index*trialDuration_s;
targetPhi=phiLevels_rad(trialId);
thetaStart=rotationDirection*2*pi*circlesPerTrial*index;
theta=thetaStart;
circleStart=phiRise_s+targetWait_s;
circleEnd=circleStart+circleDuration_s;
if local<phiRise_s
    phaseId=1;u=local/phiRise_s;phi=targetPhi*u*u*(3-2*u);
elseif local<circleStart
    phaseId=2;phi=targetPhi;
elseif local<circleEnd
    phaseId=5;direction=rotationDirection;
    elapsed=local-circleStart;
    cycleId=floor(elapsed/circleTime_s)+1;
    theta=thetaStart+rotationDirection*2*pi*elapsed/circleTime_s;
    phi=targetPhi;
elseif local<circleEnd+phiFall_s
    phaseId=3;theta=thetaStart+rotationDirection*2*pi*circlesPerTrial;
    u=(local-circleEnd)/phiFall_s;phi=targetPhi*(1-u*u*(3-2*u));
else
    phaseId=4;theta=thetaStart+rotationDirection*2*pi*circlesPerTrial;
end
end

== matlab function residual_FWD_INV_validation_v2/Seperate paramter calculation/MATLAB Function1 ==
  data: theta_des input; theta_e output; phi_e output; theta_meas input; phi_des input; phi_meas input
function [theta_e, phi_e] = configError(theta_des, theta_meas, phi_des, phi_meas)
%#codegen
% This file computes wrapped theta and phi error
%
% Inputs:
%   theta_des   : desired theta [constant] (rad)
%   theta_meas  : measured theta [constant] (rad)
%   phi_des     : desired phi [constant] (rad)
%   phi_meas    : measured phi [constant] (rad)
%
% Outputs:
%   theta_e     : bending direction [constant] (rad)
%   phi_e       : bending amount [constant] (rad)

phi_e = phi_des - phi_meas;

delta_theta = theta_des - theta_meas;
theta_e = atan2(sin(delta_theta), cos(delta_theta));

end

== matlab function residual_FWD_INV_validation_v2/helix ==
  data: t input; theta output; phi output; trialId output; phaseId output; cycleId output; direction output; done output; testEnd_s output
function [theta,phi,trialId,phaseId,cycleId,direction,done,testEnd_s] = rlHelixReferenceBlock(t)
%#codegen
% Requested theta/phi: outward then inward spiral/helix-like arm-tip path.
% Actual XYZ follows arm geometry; this is not a constant-pitch Cartesian helix.
peakPhi_rad=2.5;
circleTime_s=10.0;
turnsLoading=3;
turnsUnloading=3;
numTrials=4;
initialZero_s=5.0;
zeroHold_s=10.0;
alternateDirection=true; % CW/CCW alternate BETWEEN trials, at phi=0.
% phase: -1 invalid,0 baseline,4 zero hold,6 loading helix,
% 7 unloading helix,9 complete. Rotation does not pause at maximum phi.
assert(peakPhi_rad>=0 && peakPhi_rad<=pi && circleTime_s>0);
assert(turnsLoading>=1 && turnsLoading==floor(turnsLoading));
assert(turnsUnloading>=1 && turnsUnloading==floor(turnsUnloading));
assert(numTrials>=1 && numTrials==floor(numTrials) && initialZero_s>=0 && zeroHold_s>=0);
loading_s=turnsLoading*circleTime_s;
unloading_s=turnsUnloading*circleTime_s;
moving_s=loading_s+unloading_s;
trialDuration_s=moving_s+zeroHold_s;
turnsTotal=turnsLoading+turnsUnloading;
testEnd_s=initialZero_s+numTrials*trialDuration_s;
theta=0;phi=0;trialId=0;phaseId=0;cycleId=0;direction=0;done=false;
if ~isfinite(t) || t<0,phaseId=-1;return;end
if t<initialZero_s,return;end
if t>=testEnd_s
    turnsAccumulated=turnsTotal*numTrials;
    if alternateDirection,turnsAccumulated=turnsTotal*mod(numTrials,2);end
    theta=2*pi*turnsAccumulated;phaseId=9;done=true;return;
end
index=floor((t-initialZero_s)/trialDuration_s);
trialId=index+1;local=t-initialZero_s-index*trialDuration_s;
rotationDirection=1;turnsBefore=turnsTotal*index;
if alternateDirection
    rotationDirection=1-2*mod(index,2);
    turnsBefore=turnsTotal*mod(index,2);
end
thetaStart=2*pi*turnsBefore;
theta=thetaStart+rotationDirection*2*pi*min(local,moving_s)/circleTime_s;
if local<loading_s
    phaseId=6;direction=rotationDirection;
    cycleId=floor(local/circleTime_s)+1;
    u=local/loading_s;phi=peakPhi_rad*u*u*(3-2*u);
elseif local<moving_s
    phaseId=7;direction=rotationDirection;
    cycleId=floor(local/circleTime_s)+1;
    u=(local-loading_s)/unloading_s;
    phi=peakPhi_rad*(1-u*u*(3-2*u));
else
    phaseId=4;
end
end

== matlab function residual_FWD_INV_validation_v2/pressure combine ==
  data: t input; pressureRequest_bar output; trialId output; phaseId output; channelId output; cycleId output; done output; testEnd_s output
function [pressureRequest_bar,trialId,phaseId,channelId,cycleId,done,testEnd_s] = rlPressureCombinedBlock(t)
%#codegen
% OPEN-LOOP common/differential pressure excitation, not angle tracking.
% trialId: 1 common pulse, 2 symmetric s, 3 antisymmetric a, 4 rotating s/a.
% channelId=0 means combined channels. No deadzone compensation.
commonPeak_bar=3.0;
bias_bar=1.5;
differentialAmplitude_bar=0.5;
omega_radPerS=0.9;
cyclesPerTrial=2;
initialZero_s=5.0;
preloadRise_s=5.0;
preloadFall_s=5.0;
relax_s=10.0;
% phase: -1 invalid, 0 initial zero, 1 preload rise, 3 preload fall,
% 4 zero relaxation, 5 periodic excitation, 9 complete.
assert(commonPeak_bar>=0 && commonPeak_bar<=3 && differentialAmplitude_bar>=0);
% Conservative bound for the rotating differential combination.
assert(bias_bar-4*differentialAmplitude_bar/3>=0 && bias_bar+4*differentialAmplitude_bar/3<=3);
assert(omega_radPerS>0 && cyclesPerTrial>=1 && cyclesPerTrial==floor(cyclesPerTrial));
assert(initialZero_s>=0 && preloadRise_s>0 && preloadFall_s>0 && relax_s>0);
period_s=2*pi/omega_radPerS;
excitation_s=cyclesPerTrial*period_s;
trialDuration_s=preloadRise_s+excitation_s+preloadFall_s+relax_s;
testEnd_s=initialZero_s+4*trialDuration_s;
pressureRequest_bar=zeros(3,1);trialId=0;phaseId=0;channelId=0;cycleId=0;done=false;
if ~isfinite(t) || t<0,phaseId=-1;return;end
if t<initialZero_s,return;end
if t>=testEnd_s,phaseId=9;done=true;return;end
index=floor((t-initialZero_s)/trialDuration_s);trialId=index+1;
local=t-initialZero_s-index*trialDuration_s;
% Each mode has matching endpoints; preload/fall remove inter-mode jumps.
endpoint=zeros(3,1);
if trialId==2 || trialId==3,endpoint(:)=bias_bar;end
if trialId==4
    endpoint=[bias_bar-2*differentialAmplitude_bar/3; ...
        bias_bar+differentialAmplitude_bar/3;bias_bar+differentialAmplitude_bar/3];
end
if local<preloadRise_s
    phaseId=1;u=local/preloadRise_s;pressureRequest_bar=endpoint*u*u*(3-2*u);
elseif local<preloadRise_s+excitation_s
    phaseId=5;tau=local-preloadRise_s;angle=omega_radPerS*tau;
    cycleId=floor(tau/period_s)+1;
    if trialId==1
        pressureRequest_bar(:)=commonPeak_bar*.5*(1-cos(angle));
    else
        s=0;a=0;
        if trialId==2,s=differentialAmplitude_bar*sin(angle);end
        if trialId==3,a=differentialAmplitude_bar*sin(angle);end
        if trialId==4
            s=differentialAmplitude_bar*cos(angle);
            a=differentialAmplitude_bar*sin(angle);
        end
        pressureRequest_bar=[bias_bar-2*s/3;bias_bar+s/3-a;bias_bar+s/3+a];
    end
elseif local<preloadRise_s+excitation_s+preloadFall_s
    phaseId=3;u=(local-preloadRise_s-excitation_s)/preloadFall_s;
    pressureRequest_bar=endpoint*(1-u*u*(3-2*u));
else
    phaseId=4;
end
end

== matlab function residual_FWD_INV_validation_v2/MATLAB Function ==
  data: u input; lout output
function lout = config2length(u)
%#codegen
% Convert configuration variables to length changes
% Input (u):
%   u       : theta and phi [2x1] (rad)
%               theta angle (rad) [constant]
%               phi angle (rad) [constant]
%   r       : radial offset (m) [constant]
% 
% Output:
%   lout    : lenght changes (m) [s,1]


theta = u(1);
phi = u(2);
r = 0.013;

l = [-r * cos(theta) * phi;
    (0.5e0 * r * cos(theta) - sqrt(0.3e1) * r * sin(theta) / 0.2e1) * phi;
    (0.5e0 * r * cos(theta) + sqrt(0.3e1) * r * sin(theta) / 0.2e1) * phi];

lout = [l(2); l(3)];

end

== matlab function residual_FWD_INV_validation_v2/MATLAB Function2 ==
  data: lIn input; l output; dl output; ddl output; sampleTime_s input
function [l, dl, ddl] = lengthDerivatives(lIn, sampleTime_s)
%#codegen
% Desired reduced lengths [l2;l3] in m; derivatives in m/s and m/s^2.
% sampleTime_s is a 0.05 s zero-order-held Clock signal.
persistent lastL lastT velocity acceleration
if isempty(lastT)
    lastL = zeros(2,1);
    lastT = -1;
    velocity = zeros(2,1);
    acceleration = zeros(2,1);
end
l = lastL;
dl = velocity;
ddl = acceleration;
if ~all(isfinite(lIn)) || ~isfinite(sampleTime_s)
    return;
end
q = [lIn(1); lIn(2)];
if lastT < 0
    lastL = q;
    lastT = sampleTime_s;
    l = q;
    return;
end
dt = sampleTime_s - lastT;
if dt > 1e-6
    rawVelocity = (q-lastL)/dt;
    oldVelocity = velocity;
    alphaV = dt/(0.10+dt);
    velocity = velocity + alphaV*(rawVelocity-velocity);
    rawAcceleration = (velocity-oldVelocity)/dt;
    alphaA = dt/(0.15+dt);
    acceleration = acceleration + alphaA*(rawAcceleration-acceleration);
    lastL = q;
    lastT = sampleTime_s;
end
l = lastL;
dl = velocity;
ddl = acceleration;
end

== matlab function residual_FWD_INV_validation_v2/MATLAB Function4 ==
  settings: updateMethod=DISCRETE  sampleTime=0.05
  data: lengths3_m input; orientationValid input; predictionLength_m output double size=[2 3]; predictionAtMeasurement_m output double size=[2 3]; retimedPrediction_m output double size=[2 3]; shadowDiagnostic output Bus: ResidualShadowDiagnosticsBus size=1; inverseContext output Bus: ResidualShadowContextBus size=1; baseValid input; pollStart_s input; tipFrame input; pressure_bar input; commandTime_sim_s input; t_sim_s input; reset input; shadowOptions input
function [predictionLength_m,predictionAtMeasurement_m,retimedPrediction_m, ...
    shadowDiagnostic,inverseContext]=rlResidualShadowBlock( ...
    lengths3_m,orientationValid,baseValid,pollStart_s,tipFrame,pressure_bar, ...
    commandTime_sim_s,t_sim_s,reset,shadowOptions)
%RLRESIDUALSHADOWBLOCK Paste into a separate discrete0.05s MATLAB Function.
% Observation ONLY. Never connect any output to pressure/control/Kill inputs.
% Output columns: augmented, nominal, constant velocity. See SHADOW_VALIDATION.md.
%#codegen
persistent state
if isempty(state),state=residualShadowInitialState();end
network=residualControllerNetwork(shadowOptions(1));
[predictionLength_m,predictionAtMeasurement_m,retimedPrediction_m, ...
 shadowDiagnostic,inverseContext,state]=residualShadowStep( ...
 lengths3_m,orientationValid,baseValid,pollStart_s,tipFrame,pressure_bar, ...
 commandTime_sim_s,t_sim_s,reset,shadowOptions,state,network);
end

== matlab function residual_FWD_INV_validation_v2/MATLAB Function1 ==
  data: pressureCommand_bar input size=[3 1]; X input size=[4 1]; dX output size=[4 1]; lengths_m output size=[3 1]; theta_rad output; phi_rad output; tau_N output size=[2 1]; pressureUsed_bar output size=[3 1]; thetaObservable output; stiff input
function [dX,lengths_m,theta_rad,phi_rad,tau_N, ...
    pressureUsed_bar,thetaObservable]=rlForwardModelBlock(pressureCommand_bar,X,stiff) %#ok<INUSD>
%RLFORWARDMODELBLOCK Paste-ready nominal forward wrapper, explicit columns.
% Same3inputs/7outputs as validation-model MATLAB Function1.
% pressureCommand_bar:3 elements,bar; X:4 elements,[l2;l3;dl2;dl3].
% Original nominal constants/pressure clipping/EoM unchanged. No model I/O.
%#codegen
assert(numel(pressureCommand_bar)==3,'Pressure input must contain exactly3 elements.');
assert(numel(X)==4,'State must contain exactly4 elements.');
% Normalize at this boundary so state, torque and RHS remain column vectors.
pressureColumn=reshape(pressureCommand_bar,3,1);
stateColumn=reshape(X,4,1);
L=.17411;r=.013;mass=.1;
K=650*[2 1;1 2];D=40*eye(2);gArm=[0;0;-9.81];
mu=2000;lengthBounds=[-.035;.035;1e6];
pressureUsed_bar=min(max(pressureColumn,0),3);
forcePerBar=pi*(.013/2)^2*1e5;
% Scalar construction fixes generalized torque shape at2x1.
tau_N=[forcePerBar*(pressureUsed_bar(2)-pressureUsed_bar(1)); ...
       forcePerBar*(pressureUsed_bar(3)-pressureUsed_bar(1))];
rhs=armS_single_entry(0,stateColumn,L,r,mass,gArm,K,D,tau_N,mu,lengthBounds);
dX=[rhs(1);rhs(2);rhs(3);rhs(4)];
l2=stateColumn(1);l3=stateColumn(2);
lengths_m=[-l2-l3;l2;l3];
u=(l2+l3)/r;v=(l3-l2)/(sqrt(3)*r);
phi_rad=hypot(u,v);theta_rad=atan2(v,u);
thetaObservable=phi_rad>.5*pi/180;
end

== matlab function residual_FWD_INV_validation_v2/MATLAB Function6 ==
  settings: updateMethod=DISCRETE  sampleTime=0.05
  data: inverseContext input Bus: ResidualShadowContextBus size=1; desiredAcceleration_mPerS2 input; residualPressurePrediction_bar output double; nominalPressurePrediction_bar output double; inverseDiagnostic output Bus: ResidualShadowInverseDiagnosticsBus size=1; shadowPressureOptions input; variableCommon input; shadowInverseOptions input
function [residualPressurePrediction_bar,nominalPressurePrediction_bar,inverseDiagnostic]= ...
    rlResidualInverseShadowBlock(inverseContext,desiredAcceleration_mPerS2, ...
    shadowPressureOptions,variableCommon,shadowInverseOptions)
%RLRESIDUALINVERSESHADOWBLOCK Stateless diagnostic inverse. NO valve connection.
% Optional second block. History comes from forward observer; never commits it.
% Targets the fixed trained nominal LHS at measured q/v and supplied ddq.
% This is not PAC's adaptive/anchored control demand or a controller replacement.
%#codegen
residualPressurePrediction_bar=nan(3,1);nominalPressurePrediction_bar=nan(3,1);
inverseDiagnostic=residualShadowInverseDiagnostics();
if ~inverseContext.valid||~all(isfinite(desiredAcceleration_mPerS2)),return;end
network=residualControllerNetwork(inverseContext.units);residualValidateOptions(shadowInverseOptions);
assert(shadowInverseOptions(1)==inverseContext.units);
% Shared configuration validation only; no supervisor/anchor state is run.
cfg=residualPressureConfig(shadowPressureOptions,[0;0;1;.1;.1;1;Inf],variableCommon);
assert(abs(cfg.forcePerBar_N-network.forcePerBar)<1e-10*network.forcePerBar);
assert(cfg.activation_bar==0,'Shadow nominal reference is the training linear pressure map.');
physics=residualShadowPhysicsConfig();n=physics.nominal;
q=inverseContext.measured(1:2);v=inverseContext.measured(3:4);
P=forceResidualPhysics(q,v,n);M=[P(1),P(2);P(2),P(3)];C=[P(4),P(5);P(6),P(7)];
target=M*desiredAcceleration_mPerS2+(C+n.D)*v+n.K*q+ ...
    armS_single_boundForce(q,n.mu,n.lKbounds)+P(8:9);
step=cfg.slew_barPerS*inverseContext.horizon_s;
[nominal,~,~,nomLimited]=pacAllocatePressure(target,zeros(2,1),zeros(2,1),cfg);
nominalPressurePrediction_bar=min(max(nominal,inverseContext.pressure_bar-step),inverseContext.pressure_bar+step);
B=network.forcePerBar*[-1 1 0;-1 0 1];
[~,raw]=residualGruCell(network,[inverseContext.measured;inverseContext.pressure_bar;inverseContext.featureDt_s],inverseContext.historyPre);
[p,e,limited,iterations]=residualAllocatePressure(target,zeros(2,1),zeros(2,1),zeros(2,1), ...
    inverseContext.pressure_bar,target-raw,target,step,inverseContext.measured, ...
    inverseContext.featureDt_s,inverseContext.historyPre,network,cfg,zeros(2,1),shadowInverseOptions);
if ~all(isfinite([p;e;target])),return;end
residualPressurePrediction_bar=p;inverseDiagnostic.valid=true;
inverseDiagnostic.converged=norm(e)<=shadowInverseOptions(3);
inverseDiagnostic.limited=limited;
inverseDiagnostic.nominalLimited=nomLimited||any(abs(nominal-nominalPressurePrediction_bar)>1e-9);
inverseDiagnostic.iterations=iterations;inverseDiagnostic.targetForce_N=target;
inverseDiagnostic.predictedForce_N=target+e;inverseDiagnostic.inverseError_N=e;
inverseDiagnostic.nominalInverseError_N=B*nominalPressurePrediction_bar-target;
inverseDiagnostic.pressureDifference_bar=p-nominalPressurePrediction_bar;
inverseDiagnostic.sampleTime_host_s=inverseContext.sampleTime_host_s;
end
